simulink model "MotorXploer"  (R2026a)
settings: Solver=FixedStepAuto  StopTime=inf  FixedStep=0.001
undefined symbols (not defined in the file or in its folder): Blocking, LF, Non
libraries: fl_lib x7, amg_usbconverter_n_connect_lib x3, nesl_utility x3, dspstat3 x2
settings Model: Creator=beamk  LastModifiedBy=Legion Pro5
settings DebuggingCC: InheritedTsInSrcMsg=none

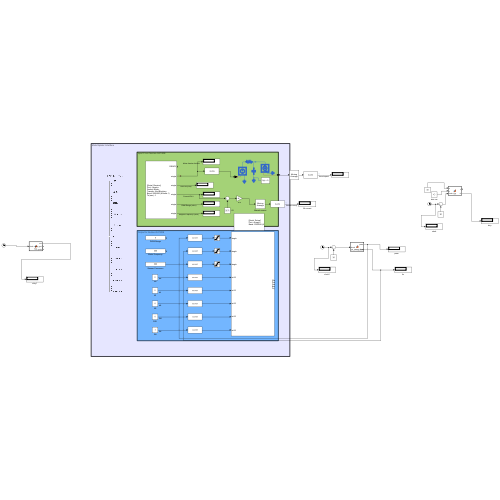
[thumbnail: Simulink's stored preview of the top-level diagram]
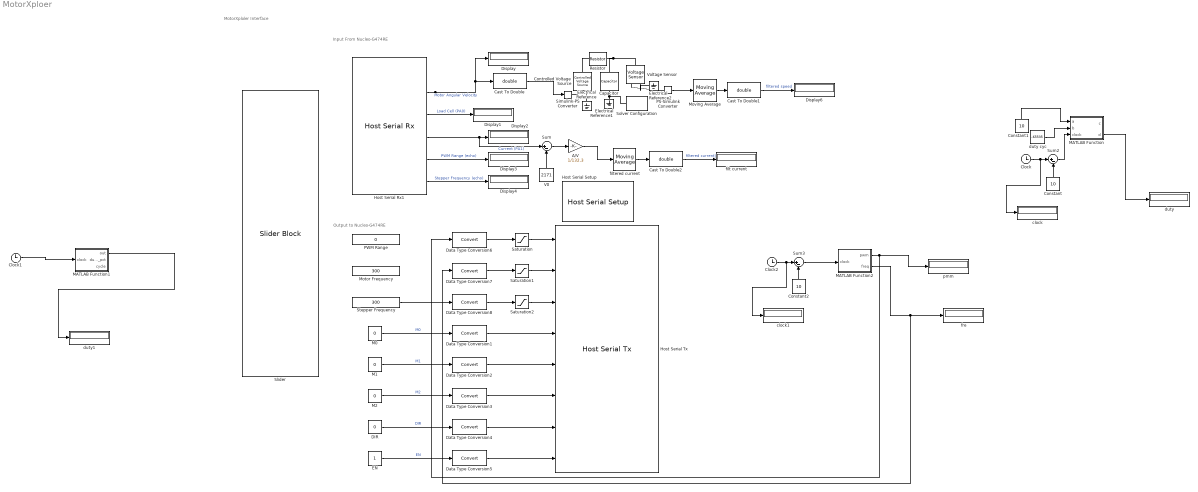
== system MotorXploer ==
  note: Output to Nucleo-G474RE
  note: Input From Nucleo-G474RE
  note: MotorXploler Interface
  A/V : Gain  Gain=1/132.3
  Capacitor : fl_lib/Electrical/Electrical Elements/Capacitor  c=470 nF  r=1e-6 Ohm  g=0 1/Ohm  i_specify=off  i_priority=None  i=0 A  i_nominal_specify=off  i_nominal_value=1  i_nominal_unit=A  v_specify=off  v_priority=None  v=0 V  v_nominal_specify=off  v_nominal_value=1  v_nominal_unit=V  vc_specify=off  vc_priority=High  vc=0 V  vc_nominal_specify=off  vc_nominal_value=1  vc_nominal_unit=V
  Cast To Double : DataTypeConversion  OutDataTypeStr=double  SaturateOnIntegerOverflow=off  RndMeth=Floor
  Cast To Double1 : DataTypeConversion  OutDataTypeStr=double  SaturateOnIntegerOverflow=off  RndMeth=Floor
  Cast To Double2 : DataTypeConversion  OutDataTypeStr=double  SaturateOnIntegerOverflow=off  RndMeth=Floor
  Clock : Clock
  Clock1 : Clock
  Clock2 : Clock
  Constant : Constant  Value=10
  Constant1 : Constant  Value=10
  Constant2 : Constant  Value=10
  Controlled Voltage Source : fl_lib/Electrical/Electrical Sources/Controlled Voltage Source
  DIR : Constant  Value=0
  Data Type Conversion{1..8} (8 alike) : DataTypeConversion  SaturateOnIntegerOverflow=off  RndMeth=Floor
  Display{,1..4,6} (6 alike) : Display
  EN : Constant
  Electrical Reference : fl_lib/Electrical/Electrical Elements/Electrical Reference
  Electrical Reference1 : fl_lib/Electrical/Electrical Elements/Electrical Reference
  Electrical Reference2 : fl_lib/Electrical/Electrical Elements/Electrical Reference
  Host Serial Rx1 : amg_usbconverter_n_connect_lib/Host Serial Rx  conf=rx  port=<auto>  baudrate=2000000  databits=8  parity=None  stopbit=1  flowcontrol=None  transfer=Non-Blocking  timeout=5  packetmode=Binary  enableinitialvalues=off  initialvalues=[]  binheader='25'  binterminator='4E'  porttype_double=0  porttype_single=5  porttype_int8=0  porttype_uint8=0  porttype_int16=0  porttype_uint16=0  porttype_int32=0  porttype_uint32=0  asciiformat='%f,%f,%d,%d'  rx_asciiterminator="LF (0x0A - \"\\n\")"  tx_asciiterminator="CRLF (0x0D 0x0A - \"\\r\\n\")"  sampletime=-1  enablecustomportlabel=off  cinputportlabel=0  coutputportlabel=A  portpinstr=0  blockid=HostSerialRx1  inputporttype=[]  inputportwidth=[]  inputportlabel={}  outputporttype=[3 1 1 1 1 1]  outputportwidth=[1 1 1 1 1 1]  outputportlabel={'READY','single','single','single','single','single'}  compat=0  optionstring=[]  autoport='<empty>'
  Host Serial Setup : amg_usbconverter_n_connect_lib/Host Serial Setup  conf=setup  port=<auto>  baudrate=2000000  databits=8  parity=None  stopbit=1  flowcontrol=None  transfer=Blocking  timeout=2  packetmode=Binary  initialvalues=[]  binheader='7E 7E'  binterminator='03 03'  porttype_double=0  porttype_single=1  porttype_int8=0  porttype_uint8=0  porttype_int16=0  porttype_uint16=0  porttype_int32=0  porttype_uint32=2  asciiformat='%d %u %x'  rx_asciiterminator="CRLF (0x0D 0x0A - \"\\r\\n\")"  tx_asciiterminator="CRLF (0x0D 0x0A - \"\\r\\n\")"  sampletime=-1  enablecustomportlabel=off  cinputportlabel=0  coutputportlabel=A  portpinstr=0  blockid=HostSerialSetup  inputporttype=[]  inputportwidth=[]  inputportlabel={}  outputporttype=[]  outputportwidth=[]  outputportlabel={}  compat=0  optionstring=[]  autoport='<empty>'
  Host Serial Tx : amg_usbconverter_n_connect_lib/Host Serial Tx  conf=tx  port=<auto>  baudrate=2000000  databits=8  parity=None  stopbit=1  flowcontrol=None  transfer=Blocking  timeout=2  packetmode=Binary  initialvalues=[]  binheader='25'  binterminator='4E'  porttype_double=0  porttype_single=3  porttype_int8=0  porttype_uint8=0  porttype_int16=5  porttype_uint16=0  porttype_int32=0  porttype_uint32=0  asciiformat='%d,%f'  rx_asciiterminator="CRLF (0x0D 0x0A - \"\\r\\n\")"  tx_asciiterminator="CRLF (0x0D 0x0A - \"\\r\\n\")"  sampletime=-1  enablecustomportlabel=off  cinputportlabel=0  coutputportlabel=A  portpinstr=0  blockid=HostSerialTx  inputporttype=[1 1 1 4 4 4 4 4]  inputportwidth=[1 1 1 1 1 1 1 1]  inputportlabel={'single','single','single','int16','int16','int16','int16','int16'}  outputporttype=[]  outputportwidth=[]  outputportlabel={}  compat=0  optionstring=[]  autoport='<empty>'
      settings: SourceProductName=aMG USB Converter N
  M0 : Constant  Value=0
  M1 : Constant  Value=0
  M2 : Constant  Value=0
  MATLAB Function : MATLAB Function  TreatAsAtomicUnit=on
  MATLAB Function1 : MATLAB Function  TreatAsAtomicUnit=on
  MATLAB Function2 : MATLAB Function  TreatAsAtomicUnit=on
  Motor Frequency : Constant  Value=300  OutDataTypeStr=single
  Moving Average : dspstat3/Moving Average  Method=Sliding window  ForgettingFactorPort=off  SpecifyWindowLength=on  WindowLengthSource=Property  MaxWindowLength=20  WindowLength=1000  OverlapLength=999  AllowArbitraryInputLength=off  ForgettingFactor=0.9  SimulateUsing=Interpreted execution
  PS-Simulink Converter : nesl_utility/PS-Simulink Converter  PhysicalDomain=network_engine_domain  SubClassName=ps_output  LeftPortType=input  RightPortType=output  PseudoPeriodic=off  Frequencies=[]  VectorFormat=inherit  Unit=inherit  AffineConversion=off
  PWM Range : Constant  Value=0  OutDataTypeStr=single
  Resistor : fl_lib/Electrical/Electrical Elements/Resistor  R=67725.5077 Ohm  i_specify=off  i_priority=None  i=0 A  i_nominal_specify=off  i_nominal_value=1  i_nominal_unit=A  v_specify=off  v_priority=None  v=0 V  v_nominal_specify=off  v_nominal_value=1  v_nominal_unit=V
  Saturation : Saturate  UpperLimit=65535  LowerLimit=-65535
  Saturation1 : Saturate  UpperLimit=20000  LowerLimit=0
  Saturation2 : Saturate  UpperLimit=inf  LowerLimit=0
  Simulink-PS Converter : nesl_utility/Simulink-PS Converter  PhysicalDomain=network_engine_domain  SubClassName=ps_input  LeftPortType=input  RightPortType=output  PseudoPeriodic=off  Frequencies=[]  NoiseDistribution=none  NoiseParameters=[]  Unit=1  AffineConversion=off  FilteringAndDerivatives=provide  SimscapeFilterOrder=1  InputFilterTimeConstant=0.001  UdotUserProvided=0
  Slider : SliderBlock  ScaleMin=-65535  ScaleMax=65535
  Solver Configuration : nesl_utility/Solver Configuration  PhysicalDomain=network_engine_domain  SubClassName=solver  LeftPortType=input  RightPortType=generic  Tones=[]  Harmonics=[]  SimulateNoise=off  Profile=off  UseLocalSampling=off  EnableSwitchedLinearOptims=on  FrequencyDomain=off  UseCCode=off  RelTol=0.001  AbsTol=0.001  MinStep=1e-09  ToWorkspace=off  RevertToSquareIcSolve=off  NumHomotopyIterations=100  PhasorMode=off  PhasorModeNumHarmonics=1  ConsistencySolver=NEWTON_XTOL_AFTER_FTOL  CanonicalOrdering=CANONICAL  OptimizeIntermediates=OPTIMIZED  IndexReductionMethod=DerivativeReplacement  DoDC=off  ResidualTolerance=1e-09  ConsistencyTolSource=GLOBAL  ConsistencyAbsTol=0.001  ConsistencyRelTol=0.001  ConsistencyTolFactor=0.001  UseLocalSolver=off  LocalSolverChoice=NE_BACKWARD_EULER_ADVANCER  ResolveIndetEquations=on  FunctionEvalNumThread=1  LocalSolverSampleTime=0.001  DoFixedCost=off  MaxNonlinIter=3  MaxModeIter=2  ComputeImpulses=off  ImpulseIterations=2  LinearAlgebra=auto  LinearAlgebraNumThread=0  EquationFormulation=NE_TIME_EF  DelaysMemoryBudget=1024  AutomaticFiltering=on  FilteringTimeConstant=0.001  PartitionStorageMethod=AS_NEEDED  PartitionMemoryBudget=1024  PartitionMethod=ROBUST  MultibodyUseLocalSolver=off  MultibodyLocalSolverChoice=ODE1  MultibodyLocalSolverSampleTime=0.001
  Stepper Frequency : Constant  Value=300  OutDataTypeStr=single
  Sum : Sum  Inputs=|+-
  Sum2 : Sum  Inputs=|+-
  Sum3 : Sum  Inputs=|+-
  V0 : Constant  Value=2171
  Voltage Sensor : fl_lib/Electrical/Electrical Sensors/Voltage Sensor
  clock : Display
  clock1 : Display
  duty : Display
  duty cyc : Constant  Value=-65535
  duty1 : Display
  filt current : Display
  filtered current : dspstat3/Moving Average  Method=Sliding window  ForgettingFactorPort=off  SpecifyWindowLength=on  WindowLengthSource=Property  MaxWindowLength=20  WindowLength=100  OverlapLength=99  AllowArbitraryInputLength=off  ForgettingFactor=0.9  SimulateUsing=Interpreted execution
  fre : Display
  pmm : Display
  wires:
  Host Serial Rx1/2 -> Display/1, Cast To Double/1  "Motor Angular Velocity"
  Host Serial Rx1/3 -> Display1/1  "Load Cell (PA0)"
  M0/1 -> Data Type Conversion1/1  "M0"
  EN/1 -> Data Type Conversion5/1  "EN"
  DIR/1 -> Data Type Conversion4/1  "DIR"
  M1/1 -> Data Type Conversion2/1  "M1"
  M2/1 -> Data Type Conversion3/1  "M2"
  Stepper Frequency/1 -> Data Type Conversion8/1
  Data Type Conversion1/1 -> Host Serial Tx/4
  Data Type Conversion2/1 -> Host Serial Tx/5
  Data Type Conversion3/1 -> Host Serial Tx/6
  Data Type Conversion4/1 -> Host Serial Tx/7
  Data Type Conversion5/1 -> Host Serial Tx/8
  Data Type Conversion6/1 -> Saturation/1
  Saturation/1 -> Host Serial Tx/1
  Data Type Conversion7/1 -> Saturation1/1
  Data Type Conversion8/1 -> Saturation2/1
  Saturation1/1 -> Host Serial Tx/2
  Saturation2/1 -> Host Serial Tx/3
  Host Serial Rx1/4 -> Sum/1, Display2/1  "Current (PA1)"
  Host Serial Rx1/5 -> Display3/1  "PWM Range (echo)"
  Host Serial Rx1/6 -> Display4/1  "Stepper Frequency (echo)"
  V0/1 -> Sum/2
  Sum/1 -> A/V/1
  A/V/1 -> filtered current/1
  Cast To Double/1 -> Simulink-PS Converter/1
  PS-Simulink Converter/1 -> Moving Average/1
  Constant/1 -> Sum2/2
  Clock/1 -> clock/1, Sum2/1
  Sum2/1 -> MATLAB Function/3(clock)
  duty cyc/1 -> MATLAB Function/2(b)
  MATLAB Function/2(d) -> duty/1
  Constant1/1 -> MATLAB Function/1(a)
  Moving Average/1 -> Cast To Double1/1
  Cast To Double1/1 -> Display6/1  "filtered speed"
  Clock1/1 -> MATLAB Function1/1(clock)
  MATLAB Function1/1(out) -> duty1/1
  Clock2/1 -> clock1/1, Sum3/1
  Constant2/1 -> Sum3/2
  Sum3/1 -> MATLAB Function2/1(clock)
  MATLAB Function2/1(pwm) -> Data Type Conversion6/1, pmm/1
  filtered current/1 -> Cast To Double2/1
  Cast To Double2/1 -> filt current/1  "filtered current]"
  MATLAB Function2/2(freq) -> Data Type Conversion7/1, fre/1
  connections:
  Simulink-PS Converter/RConn1 -- Controlled Voltage Source/RConn1
  Electrical Reference/LConn1 -- Controlled Voltage Source/RConn2
  Resistor/RConn1 -- Capacitor/LConn1 -- Voltage Sensor/LConn1
  Resistor/LConn1 -- Controlled Voltage Source/LConn1
  Electrical Reference1/LConn1 -- Solver Configuration/RConn1 -- Capacitor/RConn1
  PS-Simulink Converter/LConn1 -- Voltage Sensor/RConn1
  Voltage Sensor/RConn2 -- Electrical Reference2/LConn1

== matlab function MotorXploer/MATLAB Function1 ==
  data: clock input; out output; duty_pct output; cycle output
function [out, duty_pct, cycle] = fcn(clock)

max_val = 65535;   % +100% = full forward
min_val = -65535;  % -100% = full reverse (0 = rest)

step_time  = 2;                      % 2 seconds per 1% step
num_steps  = 201;                    % -100% to +100% inclusive = 201 steps
sweep_time = num_steps * step_time;  % 402s per sweep
wait_time  = 120;                    % 2 minutes = 120s rest at 0
cycle_time = sweep_time + wait_time; % 522s per full cycle
max_cycles = 3;

if clock < 0 || clock >= max_cycles * cycle_time
    duty_pct = 0;
    cycle = 0;
else
    cycle = floor(clock / cycle_time) + 1;
    t_in_cycle = mod(clock, cycle_time);
    
    if t_in_cycle < sweep_time
        duty_pct = -100 + floor(t_in_cycle / step_time); % -100% to +100%
    else
        duty_pct = 0;                                    % 2-minute rest at 0%
    end
end

duty = duty_pct / 100;
if duty >= 0
    out = round(duty * max_val);
else
    out = round(abs(duty) * min_val);
end
end

== matlab function MotorXploer/MATLAB Function ==
  data: a input; c output; b input; clock input; d output
function [c,d] = fcn(a,b,clock)

c = 0;
d = 0;

% --- 20% Duty Cycle (3 times) ---
if clock>=0 && clock<7
    c=0.2*a;
    d=0.2*b;
end

if clock>=7 && clock<37
    c=0;
    d=0;
end

if clock>=37 && clock<44
    c=0.2*a;
    d=0.2*b;
end

if clock>=44 && clock<74
    c=0;
    d=0;
end

if clock>=74 && clock<81
    c=0.2*a;
    d=0.2*b;
end

if clock>=81 && clock<111
    c=0;
    d=0;
end

% --- 40% Duty Cycle (3 times) ---
if clock>=111 && clock<118
    c=0.4*a;
    d=0.4*b;
end

if clock>=118 && clock<148
    c=0;
    d=0;
end

if clock>=148 && clock<155
    c=0.4*a;
    d=0.4*b;
end

if clock>=155 && clock<185
    c=0;
    d=0;
end

if clock>=185 && clock<192
    c=0.4*a;
    d=0.4*b;
end

if clock>=192 && clock<222
    c=0;
    d=0;
end

% --- 60% Duty Cycle (3 times) ---
if clock>=222 && clock<229
    c=0.6*a;
    d=0.6*b;
end

if clock>=229 && clock<259
    c=0;
    d=0;
end

if clock>=259 && clock<266
    c=0.6*a;
    d=0.6*b;
end

if clock>=266 && clock<296
    c=0;
    d=0;
end

if clock>=296 && clock<303
    c=0.6*a;
    d=0.6*b;
end

if clock>=303 && clock<333
    c=0;
    d=0;
end

% --- 80% Duty Cycle (3 times) ---
if clock>=333 && clock<340
    c=0.8*a;
    d=0.8*b;
end

if clock>=340 && clock<370
    c=0;
    d=0;
end

if clock>=370 && clock<377
    c=0.8*a;
    d=0.8*b;
end

if clock>=377 && clock<407
    c=0;
    d=0;
end

if clock>=407 && clock<414
    c=0.8*a;
    d=0.8*b;
end

if clock>=414 && clock<444
    c=0;
    d=0;
end

% --- 100% Duty Cycle (3 times) ---
if clock>=444 && clock<451
    c=a;
    d=b;
end

if clock>=451 && clock<481
    c=0;
    d=0;
end

if clock>=481 && clock<488
    c=a;
    d=b;
end

if clock>=488 && clock<518
    c=0;
    d=0;
end

if clock>=518 && clock<525
    c=a;
    d=b;
end

if clock>=525
    c=0;
    d=0;
end

== matlab function MotorXploer/MATLAB Function2 ==
  data: pwm output; clock input; freq output
function [pwm, freq] = motor_sweep_control(clock)
% MOTOR_SWEEP_CONTROL Generates PWM and frequency commands for a brushed DC motor sweep.
%
% Inputs:
%   clock - Elapsed time in seconds (scalar, starts at -10 s)
%
% Outputs:
%   pwm   - Motor PWM command (-65535 to 65535, 0 = rest)
%   freq  - PWM carrier frequency in Hz (logarithmic steps from 5 to 20000)

    % Logarithmic frequency points (Hz)
    FREQ_LIST       = [5, 10, 50, 100, 500, 1000, 5000, 10000, 20000];
    NUM_FREQ_STEPS  = length(FREQ_LIST);                 % 9 frequency levels

    % PWM sweep resolution (5% per step)
    PWM_STEP_PCT    = 0.05;
    NUM_PWM_STEPS   = round(1 / PWM_STEP_PCT) + 1;       % 21 steps (0% to 100% inclusive)

    % Single sweep configuration
    NUM_BIG_CYCLES  = 1;
    STEPS_PER_SWEEP = NUM_PWM_STEPS * NUM_FREQ_STEPS;    % 189 steps per sweep
    TOTAL_STEPS     = STEPS_PER_SWEEP * NUM_BIG_CYCLES;  % 189 total steps

    % Drive PWM limits and increment
    PWM_MIN         = -65535;
    PWM_MAX         =  65535;
    PWM_STEP        = PWM_STEP_PCT * (PWM_MAX - PWM_MIN); % 6553.5 per step

    % Timing parameters (seconds)
    T_START         = -10;                               % Pre-sweep start time
    T_SPIN          = 5;                                 % Active spin duration
    T_REST          = 10;                                % Cooldown rest duration
    T_CYCLE         = T_SPIN + T_REST;                   % 15 s total per step

    % Guard against time before -10 s or completed sweep (t >= 2835 s)
    if clock < T_START || clock >= TOTAL_STEPS * T_CYCLE
        pwm  = 0;
        freq = 0;
        return;
    end

    % Initial 10-second wait window (-10 s <= clock < 0 s): rest without shutting off PWM carrier
    if clock < 0
        pwm  = 0;
        freq = FREQ_LIST(1);                             % Hold 5 Hz ready for step 1
        return;
    end

    % Global step index (0 to 188) and elapsed time within the current 15 s step
    global_step_idx = floor(clock / T_CYCLE);
    time_in_step    = clock - (global_step_idx * T_CYCLE);

    % Step index within the sweep (0 to 188)
    sweep_step_idx  = mod(global_step_idx, STEPS_PER_SWEEP);

    % Outer loop: Frequency index (0 to 8)
    % Inner loop: PWM index (0 to 20)
    freq_idx        = floor(sweep_step_idx / NUM_PWM_STEPS);
    pwm_idx         = mod(sweep_step_idx, NUM_PWM_STEPS);

    % Look up target frequency (MATLAB uses 1-based indexing)
    freq            = FREQ_LIST(freq_idx + 1);

    % Output active PWM for the first 5 seconds, then 0 (rest) for 10 seconds
    if time_in_step < T_SPIN
        pwm = round(PWM_MIN + pwm_idx * PWM_STEP);
    else
        pwm = 0;
    end
end
